simulink subsystem "SurfEngRef"  (R2024b)
settings: Solver=VariableStepAuto  StartTime=0.0  StopTime=10.0  RelTol=1e-3
undefined symbols (not defined in the file): SimIn, SimPar
libraries: simulink x44, ServosLib x5
(part 1 of 2)
settings Model: Creator=drhill  LastModifiedBy=edison
settings SolverCC: AlgebraicLoopSolver=TrustRegion
settings OptimizationCC: ReuseModelBlockBuffer=off
settings DebuggingCC: UnconnectedInputMsg=warning  UnconnectedOutputMsg=warning  UnconnectedLineMsg=warning
settings ModelReferenceCC: EnableRefExpFcnMdlSchedulingChecks=on
settings RTWCC: GPUComputeCapability=3.5  DLArmComputeVersion=19.05

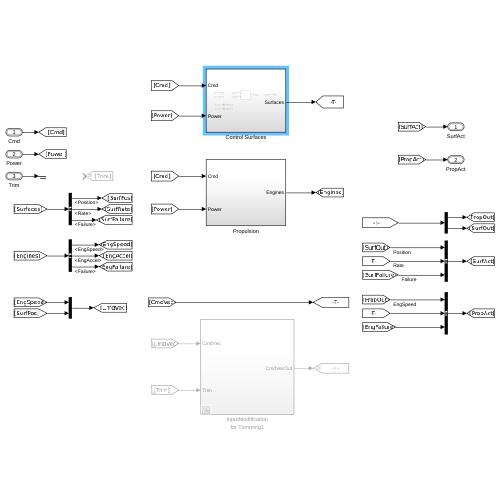
[thumbnail: Simulink's stored preview of the top-level diagram]
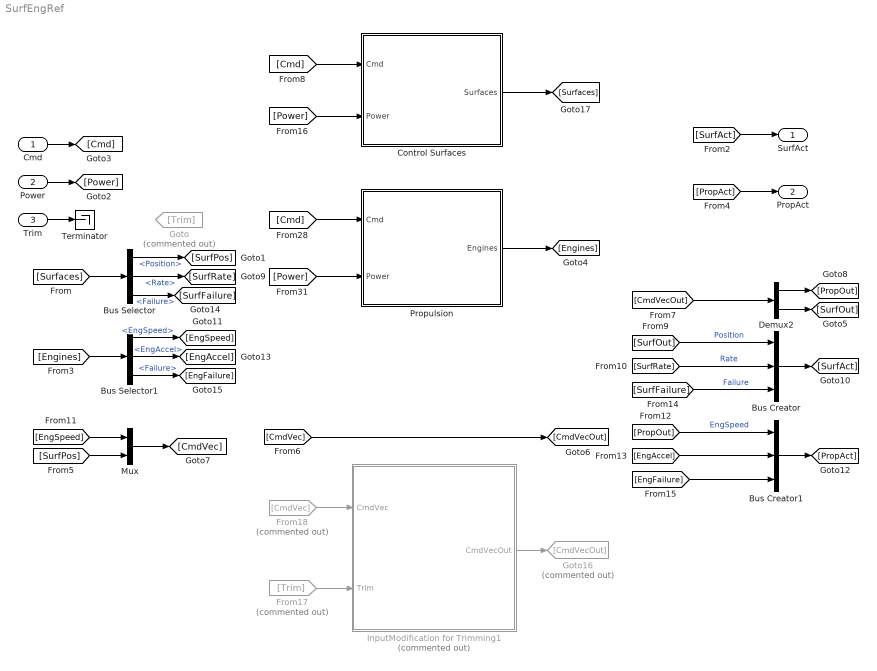
== system SurfEngRef ==
  Cmd : Inport  OutDataTypeStr=Bus: BUS_CMD
  Power : Inport  Port=2  OutDataTypeStr=Bus: BUS_POWER_SYSTEM_OUT
  Trim : Inport  Port=3  OutDataTypeStr=Bus: BUS_TRIM_INPUT
  Bus Creator : BusCreator  Inputs=3  OutDataTypeStr=Bus: BUS_SURF_ACTUATOR
  Bus Creator1 : BusCreator  Inputs=3  OutDataTypeStr=Bus: BUS_PROP_ACTUATOR
  Bus Selector : BusSelector  OutputSignals=Position,Rate,Failure
  Bus Selector1 : BusSelector  OutputSignals=EngSpeed,EngAccel,Failure
  Control Surfaces : Subsystem  VariantControl=GVS_ACT_TYPE_NONE
  Demux2 : Demux  Outputs=[SimIn.numEngines SimIn.numSurfaces]
  From17 : From  Commented=on  GotoTag=Trim
  From18 : From  Commented=on  GotoTag=CmdVec
  Goto : Goto  Commented=on  GotoTag=Trim
  Goto16 : Goto  Commented=on  GotoTag=CmdVecOut
  InputModification for Trimming1 : Subsystem  Commented=on
  Mux : Mux  Inputs=[SimIn.numEngines SimIn.numSurfaces]
  Propulsion : Subsystem  VariantControl=GVS_PROP_TYPE_NONE
  Terminator : Terminator
  SurfAct : Outport  OutDataTypeStr=Bus: BUS_SURF_ACTUATOR
  PropAct : Outport  Port=2  OutDataTypeStr=Bus: BUS_PROP_ACTUATOR
  wires:
  [Cmd] -> Control Surfaces/1(Cmd)
  [Power] -> Control Surfaces/2(Power)
  Control Surfaces/1(Surfaces) -> [Surfaces]
  Trim/1 -> Terminator/1
  Power/1 -> [Power]
  Cmd/1 -> [Cmd]
  [SurfAct] -> SurfAct/1
  [Power] -> Propulsion/2(Power)
  Propulsion/1(Engines) -> [Engines]
  [PropAct] -> PropAct/1
  [Cmd] -> Propulsion/1(Cmd)
  [CmdVec] -> [CmdVecOut]
  Mux/1 -> [CmdVec]
  [CmdVecOut] -> Demux2/1
  Demux2/2 -> [SurfOut]
  Demux2/1 -> [PropOut]
  [Surfaces] -> Bus Selector/1
  Bus Selector/1 -> [SurfPos]  "<Position>"
  [SurfPos] -> Mux/2
  [SurfOut] -> Bus Creator/1  "Position"
  Bus Selector/2 -> [SurfRate]  "<Rate>"
  [SurfRate] -> Bus Creator/2  "Rate"
  Bus Creator/1 -> [SurfAct]
  [Engines] -> Bus Selector1/1
  Bus Selector1/1 -> [EngSpeed]  "<EngSpeed>"
  [EngSpeed] -> Mux/1
  [PropOut] -> Bus Creator1/1  "EngSpeed"
  Bus Creator1/1 -> [PropAct]
  Bus Selector1/2 -> [EngAccel]  "<EngAccel>"
  [EngAccel] -> Bus Creator1/2
  Bus Selector/3 -> [SurfFailure]  "<Failure>"
  [SurfFailure] -> Bus Creator/3  "Failure"
  Bus Selector1/3 -> [EngFailure]  "<Failure>"
  [EngFailure] -> Bus Creator1/3
  InputModification for Trimming1/1(CmdVecOut) -> Goto16/1
  From18/1 -> InputModification for Trimming1/1(CmdVec)
  From17/1 -> InputModification for Trimming1/2(Trim)

== system SurfEngRef/Control Surfaces ==
  Cmd : Inport
  Power : Inport  Port=2
  Bus Selector : BusSelector  OutputSignals=CtrlSurfaceCmd
  Bus Selector1 : BusSelector  OutputSignals=CtrlSurfacePwr
  Control Surface Dynamics : Subsystem  Variant=on
  Surfaces : Outport  VectorParamsAs1DForOutWhenUnconnected=off
  wires:
  [Cmd] -> Bus Selector/1
  Bus Selector/1 -> [SurfCmd]  "<CtrlSurfaceCmd>"
  Bus Selector1/1 -> [SurfPwr]  "<CtrlSurfacePwr>"
  [Power] -> Bus Selector1/1
  [SurfPwr] -> Control Surface Dynamics/2(SurfPwr)
  Control Surface Dynamics/1(SurfAct) -> [SurfAct]
  [SurfCmd] -> Control Surface Dynamics/1(SurfCmd)
  Power/1 -> [Power]
  [SurfAct] -> Surfaces/1
  Cmd/1 -> [Cmd]

== system SurfEngRef/InputModification for Trimming1 ==
  CmdVec : Inport
  Trim : Inport  Port=2  OutDataTypeStr=Bus: BUS_TRIM_INPUT
  Constant : Constant  Value=SimIn.Switches.TrimModeOn
  "Invalid, Error Out" : Subsystem  TreatAsAtomicUnit=on
  Merge : Merge  Inputs=3  InitialOutput=zeros(SimIn.numEngines+SimIn.numSurfaces,1)
  SimMode:PassThrough : Subsystem  TreatAsAtomicUnit=on
  Switch Case : SwitchCase  CaseConditions={0,1}
  TrimMode: DriveFromTopLevel : Subsystem  TreatAsAtomicUnit=on
  CmdVecOut : Outport  VectorParamsAs1DForOutWhenUnconnected=off
  wires:
  [Trim] -> TrimMode: DriveFromTopLevel/1(TrimBias)
  [CmdVec] -> SimMode:PassThrough/1(Cmd)
  Trim/1 -> [Trim]
  CmdVec/1 -> [CmdVec]
  Switch Case/1 -> SimMode:PassThrough/Action
  Switch Case/2 -> TrimMode: DriveFromTopLevel/Action
  SimMode:PassThrough/1(Out) -> Merge/1
  TrimMode: DriveFromTopLevel/1(Out) -> Merge/2
  Merge/1 -> CmdVecOut/1
  Constant/1 -> Switch Case/1
  Switch Case/3 -> "Invalid, Error Out"/Action
  "Invalid, Error Out"/1(Out) -> Merge/3

== system SurfEngRef/Propulsion ==
  Cmd : Inport  OutDataTypeStr=Bus: BUS_CMD
  Power : Inport  Port=2
  Bus Selector : BusSelector  OutputSignals=EngineCmd
  Bus Selector1 : BusSelector  OutputSignals=EnginePwr
  Propulsion Dynamics : Subsystem  Variant=on
  Engines : Outport  OutDataTypeStr=Bus: BUS_PROP_ACTUATOR  VectorParamsAs1DForOutWhenUnconnected=off
  wires:
  Bus Selector1/1 -> [EngPwr]  "<EnginePwr>"
  [Power] -> Bus Selector1/1
  Bus Selector/1 -> [EngCmd]  "<EngineCmd>"
  [Cmd] -> Bus Selector/1
  [EngPwr] -> Propulsion Dynamics/2(EngPwr)
  [EngCmd] -> Propulsion Dynamics/1(EngCmd)
  Propulsion Dynamics/1(PropAct) -> [PropAct]
  [PropAct] -> Engines/1
  Power/1 -> [Power]
  Cmd/1 -> [Cmd]

== system SurfEngRef/Control Surfaces/Control Surface Dynamics ==
  SurfCmd : Inport
  SurfPwr : Inport  Port=2
  FirstOrder : Subsystem  VariantControl=GVS_ACT_TYPE_FIRSTORDER
  FirstOrderFailSurf : Subsystem  VariantControl=GVS_ACT_TYPE_FIRSTORDERFAILSURF
  None : Subsystem  VariantControl=GVS_ACT_TYPE_NONE
  SecondOrder : Subsystem  VariantControl=GVS_ACT_TYPE_SECONDORDER
  SurfAct : Outport

== system SurfEngRef/InputModification for Trimming1/Invalid, Error Out ==
  Action Port : ActionPort
  Constant1 : Constant  Value=zeros(SimIn.numEngines+SimIn.numSurfaces,1)
  Constant2 : Constant  Value=0
  InvalidMode : Assertion  AssertionFailFcn="warndlg('Invalid settings for TrimMode and LinearizeMode.  Run setup.m to reset.','Warning!')"
  Out : Outport  InitialOutput=zeros(SimIn.numEngines+SimIn.numSurfaces,1)  VectorParamsAs1DForOutWhenUnconnected=off
  wires:
  Constant2/1 -> InvalidMode/1
  Constant1/1 -> Out/1

== system SurfEngRef/InputModification for Trimming1/SimMode:PassThrough ==
  Cmd : Inport
  Action Port : ActionPort
  Gain1 : Gain
  Out : Outport  InitialOutput=zeros(SimIn.numEngines+SimIn.numSurfaces,1)  VectorParamsAs1DForOutWhenUnconnected=off
  wires:
  Cmd/1 -> Gain1/1  "LiftEngines(8),TailEngine,Aileron,Flaps,Elevator,Rudder"
  Gain1/1 -> Out/1

== system SurfEngRef/InputModification for Trimming1/TrimMode: DriveFromTopLevel ==
  TrimBias : Inport  OutDataTypeStr=Bus: BUS_TRIM_INPUT
  Action Port : ActionPort
  Bus Selector : BusSelector  OutputSignals=Engines,Surfaces
  Force Consistent Sample Time on Bus : Subsystem  Commented=on
  Multiply : Gain  Gain=SimIn.Trim.surfaceAlloc  Multiplication=Matrix(K*u)
  Mux : Mux  Inputs=2
  Out : Outport  InitialOutput=zeros(SimIn.numEngines+SimIn.numSurfaces,1)  VectorParamsAs1DForOutWhenUnconnected=off
  wires:
  Mux/1 -> Out/1
  Multiply/1 -> Mux/2
  Bus Selector/1 -> Mux/1  "<Engines>"
  TrimBias/1 -> Bus Selector/1
  Bus Selector/2 -> Multiply/1  "<Surfaces>"

== system SurfEngRef/Propulsion/Propulsion Dynamics ==
  EngCmd : Inport
  EngPwr : Inport  Port=2
  FirstOrder : Subsystem  VariantControl=GVS_PROP_TYPE_FIRSTORDER
  FirstOrderFailProp : Subsystem  VariantControl=GVS_PROP_TYPE_FIRSTORDERFAILPROP
  None : Subsystem  VariantControl=GVS_PROP_TYPE_NONE
  SecondOrder : Subsystem  VariantControl=GVS_PROP_TYPE_SECONDORDER
  PropAct : Outport

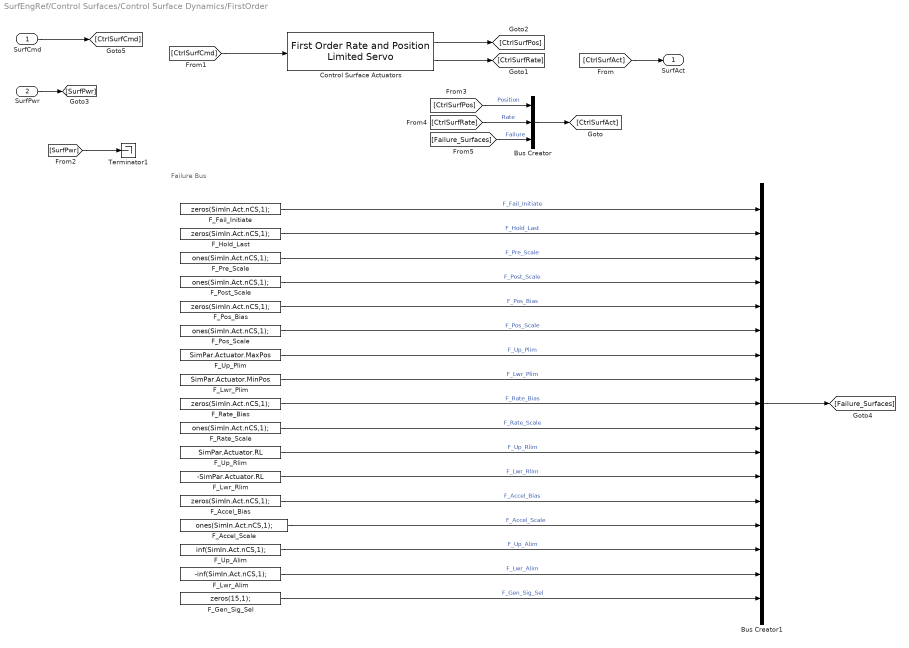
== system SurfEngRef/Control Surfaces/Control Surface Dynamics/FirstOrder ==
  note: Failure Bus
  SurfCmd : Inport
  SurfPwr : Inport  Port=2
  Bus Creator : BusCreator  Inputs=3  OutDataTypeStr=Bus: BUS_SURF_ACTUATOR
  Bus Creator1 : BusCreator  Inputs=17  OutDataTypeStr=Bus: BUS_FAILURE_SURF
  Control Surface Actuators : ServosLib/First Order  Rate and Position Limited  Servo  freq=SimPar.Actuator.BW  RL=SimPar.Actuator.RL  POS_hi=SimPar.Actuator.MaxPos  POS_lo=SimPar.Actuator.MinPos  Bias=SimPar.Actuator.Bias  StateName=Actuators
  F_Accel_Bias : Constant  Value=zeros(SimIn.Act.nCS,1);
  F_Accel_Scale : Constant  Value=ones(SimIn.Act.nCS,1);
  F_Fail_Initiate : Constant  Value=zeros(SimIn.Act.nCS,1);
  F_Gen_Sig_Sel : Constant  Value=zeros(15,1);
  F_Hold_Last : Constant  Value=zeros(SimIn.Act.nCS,1);
  F_Lwr_Alim : Constant  Value=-inf(SimIn.Act.nCS,1);
  F_Lwr_Plim : Constant  Value=SimPar.Actuator.MinPos
  F_Lwr_Rlim : Constant  Value=-SimPar.Actuator.RL
  F_Pos_Bias : Constant  Value=zeros(SimIn.Act.nCS,1);
  F_Pos_Scale : Constant  Value=ones(SimIn.Act.nCS,1);
  F_Post_Scale : Constant  Value=ones(SimIn.Act.nCS,1);
  F_Pre_Scale : Constant  Value=ones(SimIn.Act.nCS,1);
  F_Rate_Bias : Constant  Value=zeros(SimIn.Act.nCS,1);
  F_Rate_Scale : Constant  Value=ones(SimIn.Act.nCS,1);
  F_Up_Alim : Constant  Value=inf(SimIn.Act.nCS,1);
  F_Up_Plim : Constant  Value=SimPar.Actuator.MaxPos
  F_Up_Rlim : Constant  Value=SimPar.Actuator.RL
  Terminator1 : Terminator
  SurfAct : Outport
  wires:
  F_Gen_Sig_Sel/1 -> Bus Creator1/17  "F_Gen_Sig_Sel"
  F_Lwr_Alim/1 -> Bus Creator1/16  "F_Lwr_Alim"
  F_Up_Alim/1 -> Bus Creator1/15  "F_Up_Alim"
  F_Accel_Scale/1 -> Bus Creator1/14  "F_Accel_Scale"
  F_Accel_Bias/1 -> Bus Creator1/13  "F_Accel_Bias"
  F_Lwr_Rlim/1 -> Bus Creator1/12  "F_Lwr_Rlim"
  F_Up_Rlim/1 -> Bus Creator1/11  "F_Up_Rlim"
  F_Rate_Scale/1 -> Bus Creator1/10  "F_Rate_Scale"
  F_Rate_Bias/1 -> Bus Creator1/9  "F_Rate_Bias"
  F_Lwr_Plim/1 -> Bus Creator1/8  "F_Lwr_Plim"
  F_Up_Plim/1 -> Bus Creator1/7  "F_Up_Plim"
  F_Pos_Scale/1 -> Bus Creator1/6  "F_Pos_Scale"
  F_Pos_Bias/1 -> Bus Creator1/5  "F_Pos_Bias"
  F_Post_Scale/1 -> Bus Creator1/4  "F_Post_Scale"
  [Failure_Surfaces] -> Bus Creator/3  "Failure"
  F_Pre_Scale/1 -> Bus Creator1/3  "F_Pre_Scale"
  F_Hold_Last/1 -> Bus Creator1/2  "F_Hold_Last"
  Bus Creator1/1 -> [Failure_Surfaces]
  F_Fail_Initiate/1 -> Bus Creator1/1  "F_Fail_Initiate"
  [SurfPwr] -> Terminator1/1
  SurfPwr/1 -> [SurfPwr]
  SurfCmd/1 -> [CtrlSurfCmd]
  [CtrlSurfCmd] -> Control Surface Actuators/1
  Control Surface Actuators/1 -> [CtrlSurfPos]
  Control Surface Actuators/2 -> [CtrlSurfRate]
  [CtrlSurfAct] -> SurfAct/1
  [CtrlSurfPos] -> Bus Creator/1  "Position"
  [CtrlSurfRate] -> Bus Creator/2  "Rate"
  Bus Creator/1 -> [CtrlSurfAct]

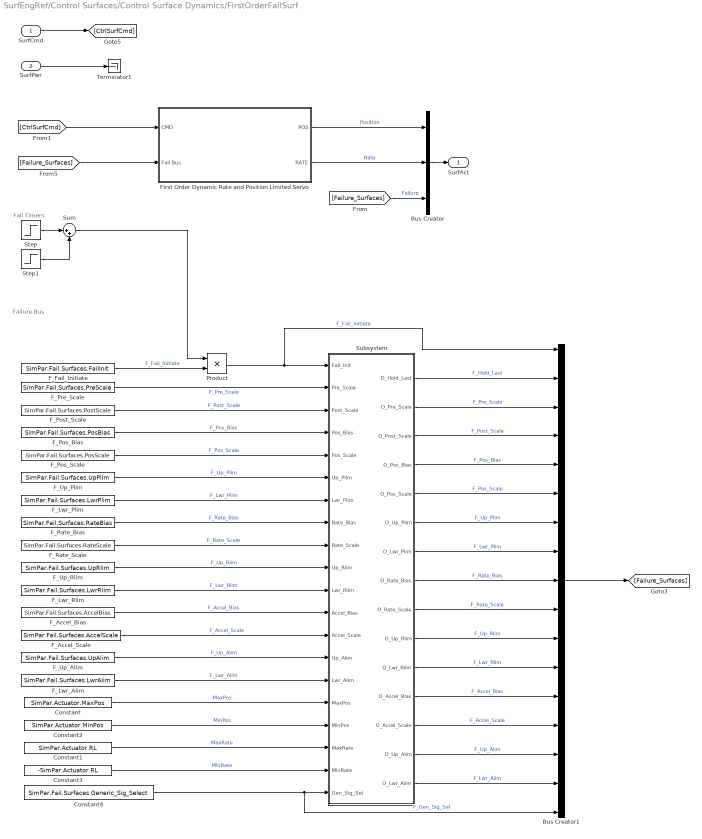
== system SurfEngRef/Control Surfaces/Control Surface Dynamics/FirstOrderFailSurf ==
  note: Failure Bus
  note: Fail Timers
  SurfCmd : Inport
  SurfPwr : Inport  Port=2
  Bus Creator : BusCreator  Inputs=3  OutDataTypeStr=Bus: BUS_SURF_ACTUATOR
  Bus Creator1 : BusCreator  Inputs=17  OutDataTypeStr=Bus: BUS_FAILURE_SURF
  Constant : Constant  Value=SimPar.Actuator.MaxPos
  Constant1 : Constant  Value=SimPar.Actuator.RL
  Constant2 : Constant  Value=SimPar.Actuator.MinPos
  Constant3 : Constant  Value=-SimPar.Actuator.RL
  Constant4 : Constant  Value=SimPar.Fail.Surfaces.Generic_Sig_Select
  F_Accel_Bias : Constant  Value=SimPar.Fail.Surfaces.AccelBias
  F_Accel_Scale : Constant  Value=SimPar.Fail.Surfaces.AccelScale
  F_Fail_Initiate : Constant  Value=SimPar.Fail.Surfaces.FailInit
  F_Lwr_Alim : Constant  Value=SimPar.Fail.Surfaces.LwrAlim
  F_Lwr_Plim : Constant  Value=SimPar.Fail.Surfaces.LwrPlim
  F_Lwr_Rlim : Constant  Value=SimPar.Fail.Surfaces.LwrRlim
  F_Pos_Bias : Constant  Value=SimPar.Fail.Surfaces.PosBias
  F_Pos_Scale : Constant  Value=SimPar.Fail.Surfaces.PosScale
  F_Post_Scale : Constant  Value=SimPar.Fail.Surfaces.PostScale
  F_Pre_Scale : Constant  Value=SimPar.Fail.Surfaces.PreScale
  F_Rate_Bias : Constant  Value=SimPar.Fail.Surfaces.RateBias
  F_Rate_Scale : Constant  Value=SimPar.Fail.Surfaces.RateScale
  F_Up_Alim : Constant  Value=SimPar.Fail.Surfaces.UpAlim
  F_Up_Plim : Constant  Value=SimPar.Fail.Surfaces.UpPlim
  F_Up_Rlim : Constant  Value=SimPar.Fail.Surfaces.UpRlim
  First Order Dynamic Rate and Position Limited Servo : Subsystem  AncestorBlock=ServosLib/First Order Dynamic Rate and Position Limited Servo  mask(Rate and Position Limited Servo){freq=SimPar.Actuator.BW, Bias=SimPar.Actuator.Bias, StateName='Actuators'}
      mask prompts: freq "Bandwidth, Hz:"; Bias "Bias Value, rad:"; StateName "State Name:"
      mask help: First order transfer function: w/(s+w), with rate and position limits and output bias level.
      mask init:
      | %omega=2*pi*freq;
      mask Display:
      | text(.48,.70,'1st Order','horizontalAlignment','center');
      | text(.48,.50,'Rate and Position Limited','horizontalAlignment','center');
      | text(.48,.30,'Filter','horizontalAlignment','center');
  Product : Product
  Step : Step  Time=SimPar.Fail.Surfaces.InitTime  SampleTime=0
  Step1 : Step  Time=SimPar.Fail.Surfaces.StopTime  After=-1  SampleTime=0
  Subsystem : Subsystem
  Sum : Sum  Inputs=|++
  Terminator1 : Terminator
  SurfAct : Outport
  wires:
  [Failure_Surfaces] -> Bus Creator/3  "Failure"
  Constant4/1 -> Bus Creator1/17, Subsystem/20(Gen_Sig_Sel)  "F_Gen_Sig_Sel"
  Sum/1 -> Product/1
  Product/1 -> Subsystem/1(Fail_Init), Bus Creator1/1  "F_Fail_Initiate"
  Step1/1 -> Sum/2
  Step/1 -> Sum/1
  Subsystem/13(O_Accel_Scale) -> Bus Creator1/14  "F_Accel_Scale"
  Subsystem/12(O_Accel_Bias) -> Bus Creator1/13  "F_Accel_Bias"
  Subsystem/15(O_Lwr_Alim) -> Bus Creator1/16  "F_Lwr_Alim"
  Subsystem/14(O_Up_Alim) -> Bus Creator1/15  "F_Up_Alim"
  Subsystem/11(O_Lwr_Rlim) -> Bus Creator1/12  "F_Lwr_Rlim"
  Subsystem/10(O_Up_Rlim) -> Bus Creator1/11  "F_Up_Rlim"
  Subsystem/9(O_Rate_Scale) -> Bus Creator1/10  "F_Rate_Scale"
  Subsystem/8(O_Rate_Bias) -> Bus Creator1/9  "F_Rate_Bias"
  Subsystem/7(O_Lwr_Plim) -> Bus Creator1/8  "F_Lwr_Plim"
  Subsystem/6(O_Up_Plim) -> Bus Creator1/7  "F_Up_Plim"
  Subsystem/5(O_Pos_Scale) -> Bus Creator1/6  "F_Pos_Scale"
  Subsystem/4(O_Pos_Bias) -> Bus Creator1/5  "F_Pos_Bias"
  Subsystem/3(O_Post_Scale) -> Bus Creator1/4  "F_Post_Scale"
  Subsystem/2(O_Pre_Scale) -> Bus Creator1/3  "F_Pre_Scale"
  Subsystem/1(O_Hold_Last) -> Bus Creator1/2  "F_Hold_Last"
  Bus Creator1/1 -> [Failure_Surfaces]
  F_Post_Scale/1 -> Subsystem/3(Post_Scale)  "F_Post_Scale"
  F_Accel_Scale/1 -> Subsystem/13(Accel_Scale)  "F_Accel_Scale"
  F_Lwr_Alim/1 -> Subsystem/15(Lwr_Alim)  "F_Lwr_Alim"
  [Failure_Surfaces] -> First Order Dynamic Rate and Position Limited Servo/2(Fail Bus)
  [CtrlSurfCmd] -> First Order Dynamic Rate and Position Limited Servo/1(CMD)
  First Order Dynamic Rate and Position Limited Servo/2(RATE) -> Bus Creator/2  "Rate"
  F_Lwr_Plim/1 -> Subsystem/7(Lwr_Plim)  "F_Lwr_Plim"
  F_Up_Plim/1 -> Subsystem/6(Up_Plim)  "F_Up_Plim"
  F_Pos_Bias/1 -> Subsystem/4(Pos_Bias)  "F_Pos_Bias"
  F_Rate_Bias/1 -> Subsystem/8(Rate_Bias)  "F_Rate_Bias"
  F_Lwr_Rlim/1 -> Subsystem/11(Lwr_Rlim)  "F_Lwr_Rlim"
  F_Fail_Initiate/1 -> Product/2  "F_Fail_Initiate"
  SurfPwr/1 -> Terminator1/1
  Constant1/1 -> Subsystem/18(MaxRate)  "MaxRate"
  Constant3/1 -> Subsystem/19(MinRate)  "MinRate"
  F_Pos_Scale/1 -> Subsystem/5(Pos_Scale)  "F_Pos_Scale"
  Bus Creator/1 -> SurfAct/1
  Constant2/1 -> Subsystem/17(MinPos)  "MinPos"
  Constant/1 -> Subsystem/16(MaxPos)  "MaxPos"
  F_Pre_Scale/1 -> Subsystem/2(Pre_Scale)  "F_Pre_Scale"
  F_Up_Alim/1 -> Subsystem/14(Up_Alim)  "F_Up_Alim"
  F_Rate_Scale/1 -> Subsystem/9(Rate_Scale)  "F_Rate_Scale"
  F_Accel_Bias/1 -> Subsystem/12(Accel_Bias)  "F_Accel_Bias"
  SurfCmd/1 -> [CtrlSurfCmd]
  F_Up_Rlim/1 -> Subsystem/10(Up_Rlim)  "F_Up_Rlim"
  First Order Dynamic Rate and Position Limited Servo/1(POS) -> Bus Creator/1  "Position"

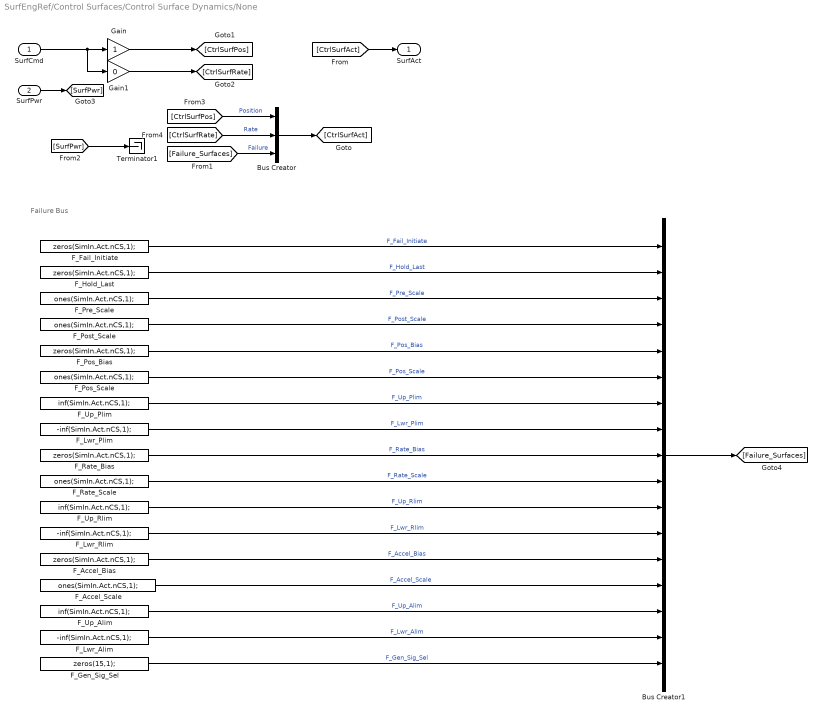
== system SurfEngRef/Control Surfaces/Control Surface Dynamics/None ==
  note: Failure Bus
  SurfCmd : Inport
  SurfPwr : Inport  Port=2
  Bus Creator : BusCreator  Inputs=3  OutDataTypeStr=Bus: BUS_SURF_ACTUATOR
  Bus Creator1 : BusCreator  Inputs=17  OutDataTypeStr=Bus: BUS_FAILURE_SURF
  F_Accel_Bias : Constant  Value=zeros(SimIn.Act.nCS,1);
  F_Accel_Scale : Constant  Value=ones(SimIn.Act.nCS,1);
  F_Fail_Initiate : Constant  Value=zeros(SimIn.Act.nCS,1);
  F_Gen_Sig_Sel : Constant  Value=zeros(15,1);
  F_Hold_Last : Constant  Value=zeros(SimIn.Act.nCS,1);
  F_Lwr_Alim : Constant  Value=-inf(SimIn.Act.nCS,1);
  F_Lwr_Plim : Constant  Value=-inf(SimIn.Act.nCS,1);
  F_Lwr_Rlim : Constant  Value=-inf(SimIn.Act.nCS,1);
  F_Pos_Bias : Constant  Value=zeros(SimIn.Act.nCS,1);
  F_Pos_Scale : Constant  Value=ones(SimIn.Act.nCS,1);
  F_Post_Scale : Constant  Value=ones(SimIn.Act.nCS,1);
  F_Pre_Scale : Constant  Value=ones(SimIn.Act.nCS,1);
  F_Rate_Bias : Constant  Value=zeros(SimIn.Act.nCS,1);
  F_Rate_Scale : Constant  Value=ones(SimIn.Act.nCS,1);
  F_Up_Alim : Constant  Value=inf(SimIn.Act.nCS,1);
  F_Up_Plim : Constant  Value=inf(SimIn.Act.nCS,1);
  F_Up_Rlim : Constant  Value=inf(SimIn.Act.nCS,1);
  Gain : Gain
  Gain1 : Gain  Gain=0
  Terminator1 : Terminator
  SurfAct : Outport
  wires:
  F_Gen_Sig_Sel/1 -> Bus Creator1/17  "F_Gen_Sig_Sel"
  F_Lwr_Alim/1 -> Bus Creator1/16  "F_Lwr_Alim"
  F_Up_Alim/1 -> Bus Creator1/15  "F_Up_Alim"
  F_Accel_Scale/1 -> Bus Creator1/14  "F_Accel_Scale"
  F_Accel_Bias/1 -> Bus Creator1/13  "F_Accel_Bias"
  F_Lwr_Rlim/1 -> Bus Creator1/12  "F_Lwr_Rlim"
  F_Up_Rlim/1 -> Bus Creator1/11  "F_Up_Rlim"
  F_Rate_Scale/1 -> Bus Creator1/10  "F_Rate_Scale"
  F_Rate_Bias/1 -> Bus Creator1/9  "F_Rate_Bias"
  F_Lwr_Plim/1 -> Bus Creator1/8  "F_Lwr_Plim"
  F_Up_Plim/1 -> Bus Creator1/7  "F_Up_Plim"
  F_Pos_Scale/1 -> Bus Creator1/6  "F_Pos_Scale"
  F_Pos_Bias/1 -> Bus Creator1/5  "F_Pos_Bias"
  F_Post_Scale/1 -> Bus Creator1/4  "F_Post_Scale"
  F_Pre_Scale/1 -> Bus Creator1/3  "F_Pre_Scale"
  [Failure_Surfaces] -> Bus Creator/3  "Failure"
  F_Fail_Initiate/1 -> Bus Creator1/1  "F_Fail_Initiate"
  Bus Creator1/1 -> [Failure_Surfaces]
  F_Hold_Last/1 -> Bus Creator1/2  "F_Hold_Last"
  Gain1/1 -> [CtrlSurfRate]
  Gain/1 -> [CtrlSurfPos]
  [CtrlSurfAct] -> SurfAct/1
  [CtrlSurfRate] -> Bus Creator/2  "Rate"
  [CtrlSurfPos] -> Bus Creator/1  "Position"
  Bus Creator/1 -> [CtrlSurfAct]
  [SurfPwr] -> Terminator1/1
  SurfPwr/1 -> [SurfPwr]
  SurfCmd/1 -> Gain1/1, Gain/1

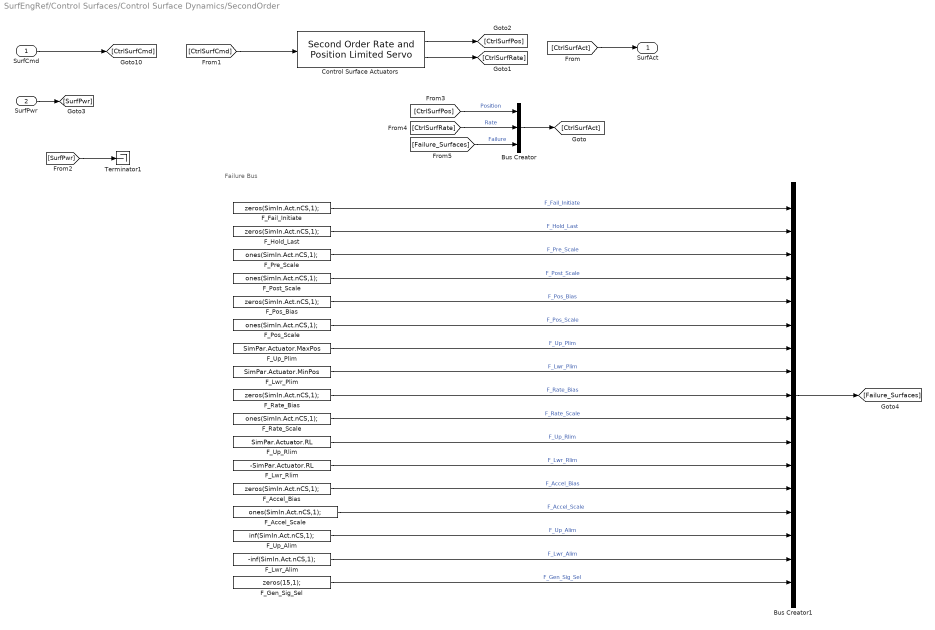
== system SurfEngRef/Control Surfaces/Control Surface Dynamics/SecondOrder ==
  note: Failure Bus
  SurfCmd : Inport
  SurfPwr : Inport  Port=2
  Bus Creator : BusCreator  Inputs=3  OutDataTypeStr=Bus: BUS_SURF_ACTUATOR
  Bus Creator1 : BusCreator  Inputs=17  OutDataTypeStr=Bus: BUS_FAILURE_SURF
  Control Surface Actuators : ServosLib/Second Order Rate and Position Limited Servo  freq=SimPar.Actuator.BW  zeta=SimPar.Actuator.Zeta  RL=SimPar.Actuator.RL  POS_hi=SimPar.Actuator.MaxPos  POS_lo=SimPar.Actuator.MinPos  Bias=SimPar.Actuator.Bias  PosStateName=ActuatorPosition  RateStateName=ActuatorRate
  F_Accel_Bias : Constant  Value=zeros(SimIn.Act.nCS,1);
  F_Accel_Scale : Constant  Value=ones(SimIn.Act.nCS,1);
  F_Fail_Initiate : Constant  Value=zeros(SimIn.Act.nCS,1);
  F_Gen_Sig_Sel : Constant  Value=zeros(15,1);
  F_Hold_Last : Constant  Value=zeros(SimIn.Act.nCS,1);
  F_Lwr_Alim : Constant  Value=-inf(SimIn.Act.nCS,1);
  F_Lwr_Plim : Constant  Value=SimPar.Actuator.MinPos
  F_Lwr_Rlim : Constant  Value=-SimPar.Actuator.RL
  F_Pos_Bias : Constant  Value=zeros(SimIn.Act.nCS,1);
  F_Pos_Scale : Constant  Value=ones(SimIn.Act.nCS,1);
  F_Post_Scale : Constant  Value=ones(SimIn.Act.nCS,1);
  F_Pre_Scale : Constant  Value=ones(SimIn.Act.nCS,1);
  F_Rate_Bias : Constant  Value=zeros(SimIn.Act.nCS,1);
  F_Rate_Scale : Constant  Value=ones(SimIn.Act.nCS,1);
  F_Up_Alim : Constant  Value=inf(SimIn.Act.nCS,1);
  F_Up_Plim : Constant  Value=SimPar.Actuator.MaxPos
  F_Up_Rlim : Constant  Value=SimPar.Actuator.RL
  Terminator1 : Terminator
  SurfAct : Outport
  wires:
  F_Lwr_Alim/1 -> Bus Creator1/16  "F_Lwr_Alim"
  F_Rate_Scale/1 -> Bus Creator1/10  "F_Rate_Scale"
  F_Rate_Bias/1 -> Bus Creator1/9  "F_Rate_Bias"
  F_Post_Scale/1 -> Bus Creator1/4  "F_Post_Scale"
  F_Up_Rlim/1 -> Bus Creator1/11  "F_Up_Rlim"
  F_Lwr_Rlim/1 -> Bus Creator1/12  "F_Lwr_Rlim"
  F_Hold_Last/1 -> Bus Creator1/2  "F_Hold_Last"
  F_Lwr_Plim/1 -> Bus Creator1/8  "F_Lwr_Plim"
  F_Accel_Bias/1 -> Bus Creator1/13  "F_Accel_Bias"
  F_Gen_Sig_Sel/1 -> Bus Creator1/17  "F_Gen_Sig_Sel"
  F_Accel_Scale/1 -> Bus Creator1/14  "F_Accel_Scale"
  F_Up_Alim/1 -> Bus Creator1/15  "F_Up_Alim"
  F_Pre_Scale/1 -> Bus Creator1/3  "F_Pre_Scale"
  F_Up_Plim/1 -> Bus Creator1/7  "F_Up_Plim"
  F_Pos_Bias/1 -> Bus Creator1/5  "F_Pos_Bias"
  F_Pos_Scale/1 -> Bus Creator1/6  "F_Pos_Scale"
  F_Fail_Initiate/1 -> Bus Creator1/1  "F_Fail_Initiate"
  Bus Creator1/1 -> [Failure_Surfaces]
  [Failure_Surfaces] -> Bus Creator/3  "Failure"
  [CtrlSurfRate] -> Bus Creator/2  "Rate"
  [CtrlSurfPos] -> Bus Creator/1  "Position"
  Bus Creator/1 -> [CtrlSurfAct]
  Control Surface Actuators/2 -> [CtrlSurfRate]
  Control Surface Actuators/1 -> [CtrlSurfPos]
  [SurfPwr] -> Terminator1/1
  SurfCmd/1 -> [CtrlSurfCmd]
  [CtrlSurfCmd] -> Control Surface Actuators/1
  [CtrlSurfAct] -> SurfAct/1
  SurfPwr/1 -> [SurfPwr]

== system SurfEngRef/InputModification for Trimming1/TrimMode: DriveFromTopLevel/Force Consistent Sample Time on Bus ==
  TrimBias : Inport
  Bus to Vector : BusToVector
  Map4 : Gain
  Out1 : Outport  VectorParamsAs1DForOutWhenUnconnected=off
  wires:
  Bus to Vector/1 -> Map4/1
  Map4/1 -> Out1/1
  TrimBias/1 -> Bus to Vector/1

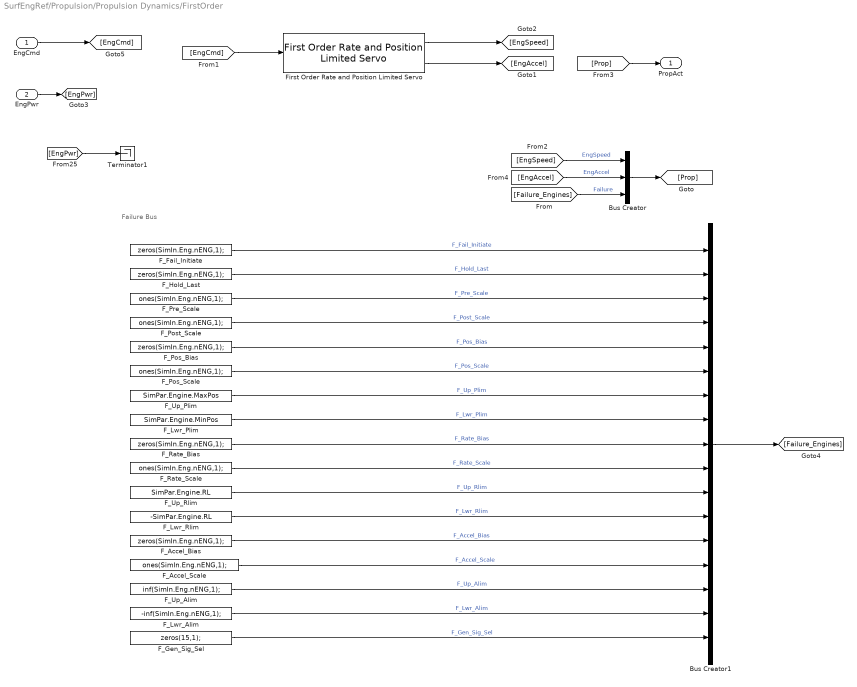
== system SurfEngRef/Propulsion/Propulsion Dynamics/FirstOrder ==
  note: Failure Bus
  EngCmd : Inport
  EngPwr : Inport  Port=2
  Bus Creator : BusCreator  Inputs=3  OutDataTypeStr=Bus: BUS_PROP_ACTUATOR
  Bus Creator1 : BusCreator  Inputs=17  OutDataTypeStr=Bus: BUS_FAILURE_ENG
  F_Accel_Bias : Constant  Value=zeros(SimIn.Eng.nENG,1);
  F_Accel_Scale : Constant  Value=ones(SimIn.Eng.nENG,1);
  F_Fail_Initiate : Constant  Value=zeros(SimIn.Eng.nENG,1);
  F_Gen_Sig_Sel : Constant  Value=zeros(15,1);
  F_Hold_Last : Constant  Value=zeros(SimIn.Eng.nENG,1);
  F_Lwr_Alim : Constant  Value=-inf(SimIn.Eng.nENG,1);
  F_Lwr_Plim : Constant  Value=SimPar.Engine.MinPos
  F_Lwr_Rlim : Constant  Value=-SimPar.Engine.RL
  F_Pos_Bias : Constant  Value=zeros(SimIn.Eng.nENG,1);
  F_Pos_Scale : Constant  Value=ones(SimIn.Eng.nENG,1);
  F_Post_Scale : Constant  Value=ones(SimIn.Eng.nENG,1);
  F_Pre_Scale : Constant  Value=ones(SimIn.Eng.nENG,1);
  F_Rate_Bias : Constant  Value=zeros(SimIn.Eng.nENG,1);
  F_Rate_Scale : Constant  Value=ones(SimIn.Eng.nENG,1);
  F_Up_Alim : Constant  Value=inf(SimIn.Eng.nENG,1);
  F_Up_Plim : Constant  Value=SimPar.Engine.MaxPos
  F_Up_Rlim : Constant  Value=SimPar.Engine.RL
  First Order Rate and Position Limited Servo : ServosLib/First Order  Rate and Position Limited  Servo  freq=SimPar.Engine.BW  RL=SimPar.Engine.RL  POS_hi=SimPar.Engine.MaxPos  POS_lo=SimPar.Engine.MinPos  Bias=SimPar.Engine.Bias  StateName=EngineSpeed
  Terminator1 : Terminator
  PropAct : Outport
  wires:
  [Failure_Engines] -> Bus Creator/3  "Failure"
  F_Lwr_Alim/1 -> Bus Creator1/16  "F_Lwr_Alim"
  F_Rate_Scale/1 -> Bus Creator1/10  "F_Rate_Scale"
  F_Rate_Bias/1 -> Bus Creator1/9  "F_Rate_Bias"
  F_Post_Scale/1 -> Bus Creator1/4  "F_Post_Scale"
  F_Up_Rlim/1 -> Bus Creator1/11  "F_Up_Rlim"
  F_Lwr_Rlim/1 -> Bus Creator1/12  "F_Lwr_Rlim"
  F_Hold_Last/1 -> Bus Creator1/2  "F_Hold_Last"
  F_Lwr_Plim/1 -> Bus Creator1/8  "F_Lwr_Plim"
  F_Accel_Bias/1 -> Bus Creator1/13  "F_Accel_Bias"
  F_Gen_Sig_Sel/1 -> Bus Creator1/17  "F_Gen_Sig_Sel"
  F_Accel_Scale/1 -> Bus Creator1/14  "F_Accel_Scale"
  F_Up_Alim/1 -> Bus Creator1/15  "F_Up_Alim"
  F_Pre_Scale/1 -> Bus Creator1/3  "F_Pre_Scale"
  F_Up_Plim/1 -> Bus Creator1/7  "F_Up_Plim"
  F_Pos_Bias/1 -> Bus Creator1/5  "F_Pos_Bias"
  F_Pos_Scale/1 -> Bus Creator1/6  "F_Pos_Scale"
  F_Fail_Initiate/1 -> Bus Creator1/1  "F_Fail_Initiate"
  Bus Creator1/1 -> [Failure_Engines]
  First Order Rate and Position Limited Servo/2 -> [EngAccel]
  First Order Rate and Position Limited Servo/1 -> [EngSpeed]
  [Prop] -> PropAct/1
  [EngPwr] -> Terminator1/1
  [EngCmd] -> First Order Rate and Position Limited Servo/1
  EngPwr/1 -> [EngPwr]
  EngCmd/1 -> [EngCmd]
  [EngSpeed] -> Bus Creator/1  "EngSpeed"
  Bus Creator/1 -> [Prop]
  [EngAccel] -> Bus Creator/2  "EngAccel"

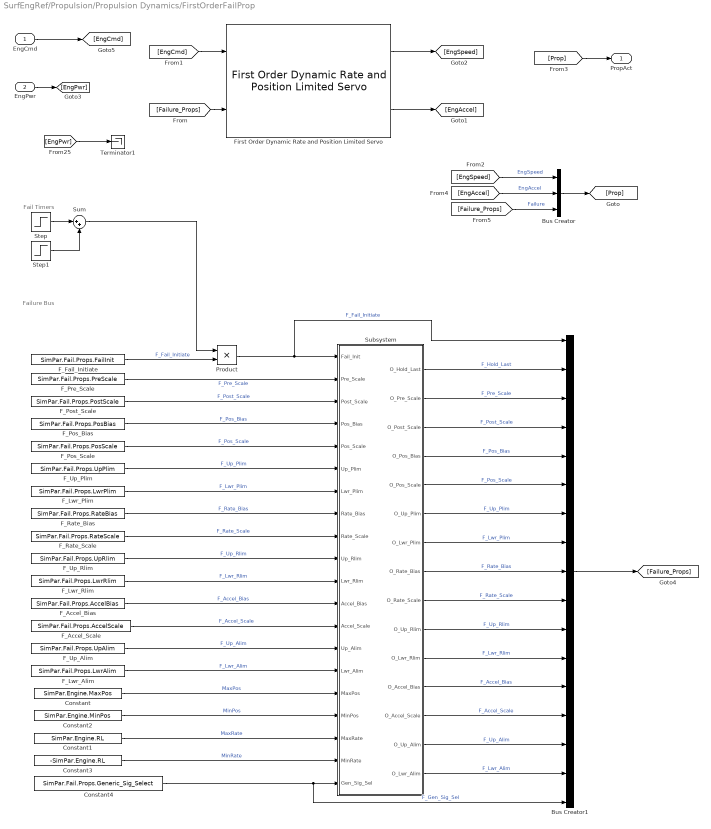
== system SurfEngRef/Propulsion/Propulsion Dynamics/FirstOrderFailProp ==
  note: Failure Bus
  note: Fail Timers
  EngCmd : Inport
  EngPwr : Inport  Port=2
  Bus Creator : BusCreator  Inputs=3  OutDataTypeStr=Bus: BUS_PROP_ACTUATOR
  Bus Creator1 : BusCreator  Inputs=17  OutDataTypeStr=Bus: BUS_FAILURE_ENG
  Constant : Constant  Value=SimPar.Engine.MaxPos
  Constant1 : Constant  Value=SimPar.Engine.RL
  Constant2 : Constant  Value=SimPar.Engine.MinPos
  Constant3 : Constant  Value=-SimPar.Engine.RL
  Constant4 : Constant  Value=SimPar.Fail.Props.Generic_Sig_Select
  F_Accel_Bias : Constant  Value=SimPar.Fail.Props.AccelBias
  F_Accel_Scale : Constant  Value=SimPar.Fail.Props.AccelScale
  F_Fail_Initiate : Constant  Value=SimPar.Fail.Props.FailInit
  F_Lwr_Alim : Constant  Value=SimPar.Fail.Props.LwrAlim
  F_Lwr_Plim : Constant  Value=SimPar.Fail.Props.LwrPlim
  F_Lwr_Rlim : Constant  Value=SimPar.Fail.Props.LwrRlim
  F_Pos_Bias : Constant  Value=SimPar.Fail.Props.PosBias
  F_Pos_Scale : Constant  Value=SimPar.Fail.Props.PosScale
  F_Post_Scale : Constant  Value=SimPar.Fail.Props.PostScale
  F_Pre_Scale : Constant  Value=SimPar.Fail.Props.PreScale
  F_Rate_Bias : Constant  Value=SimPar.Fail.Props.RateBias
  F_Rate_Scale : Constant  Value=SimPar.Fail.Props.RateScale
  F_Up_Alim : Constant  Value=SimPar.Fail.Props.UpAlim
  F_Up_Plim : Constant  Value=SimPar.Fail.Props.UpPlim
  F_Up_Rlim : Constant  Value=SimPar.Fail.Props.UpRlim
  First Order Dynamic Rate and Position Limited Servo : ServosLib/First Order Dynamic Rate and Position Limited Servo  freq=SimPar.Engine.BW  Bias=SimPar.Engine.Bias  StateName='Engines'
  Product : Product
  Step : Step  Time=SimPar.Fail.Props.InitTime  SampleTime=0
  Step1 : Step  Time=SimPar.Fail.Props.StopTime  After=-1  SampleTime=0
  Subsystem : Subsystem
  Sum : Sum  Inputs=|++
  Terminator1 : Terminator
  PropAct : Outport
  wires:
  [EngPwr] -> Terminator1/1
  [EngAccel] -> Bus Creator/2  "EngAccel"
  Bus Creator/1 -> [Prop]
  First Order Dynamic Rate and Position Limited Servo/2 -> [EngAccel]
  [Prop] -> PropAct/1
  [EngSpeed] -> Bus Creator/1  "EngSpeed"
  EngPwr/1 -> [EngPwr]
  EngCmd/1 -> [EngCmd]
  [EngCmd] -> First Order Dynamic Rate and Position Limited Servo/1
  First Order Dynamic Rate and Position Limited Servo/1 -> [EngSpeed]
  F_Up_Rlim/1 -> Subsystem/10(Up_Rlim)  "F_Up_Rlim"
  Subsystem/4(O_Pos_Bias) -> Bus Creator1/5  "F_Pos_Bias"
  F_Accel_Bias/1 -> Subsystem/12(Accel_Bias)  "F_Accel_Bias"
  Subsystem/11(O_Lwr_Rlim) -> Bus Creator1/12  "F_Lwr_Rlim"
  F_Pos_Bias/1 -> Subsystem/4(Pos_Bias)  "F_Pos_Bias"
  F_Rate_Bias/1 -> Subsystem/8(Rate_Bias)  "F_Rate_Bias"
  Constant2/1 -> Subsystem/17(MinPos)  "MinPos"
  F_Up_Alim/1 -> Subsystem/14(Up_Alim)  "F_Up_Alim"
  Product/1 -> Subsystem/1(Fail_Init), Bus Creator1/1  "F_Fail_Initiate"
  F_Pre_Scale/1 -> Subsystem/2(Pre_Scale)  "F_Pre_Scale"
  F_Pos_Scale/1 -> Subsystem/5(Pos_Scale)  "F_Pos_Scale"
  F_Fail_Initiate/1 -> Product/2  "F_Fail_Initiate"
  Subsystem/13(O_Accel_Scale) -> Bus Creator1/14  "F_Accel_Scale"
  F_Rate_Scale/1 -> Subsystem/9(Rate_Scale)  "F_Rate_Scale"
  Constant1/1 -> Subsystem/18(MaxRate)  "MaxRate"
  F_Lwr_Rlim/1 -> Subsystem/11(Lwr_Rlim)  "F_Lwr_Rlim"
  F_Lwr_Plim/1 -> Subsystem/7(Lwr_Plim)  "F_Lwr_Plim"
  Subsystem/12(O_Accel_Bias) -> Bus Creator1/13  "F_Accel_Bias"
  Constant3/1 -> Subsystem/19(MinRate)  "MinRate"
  Subsystem/5(O_Pos_Scale) -> Bus Creator1/6  "F_Pos_Scale"
  Subsystem/2(O_Pre_Scale) -> Bus Creator1/3  "F_Pre_Scale"
  Subsystem/7(O_Lwr_Plim) -> Bus Creator1/8  "F_Lwr_Plim"
  F_Accel_Scale/1 -> Subsystem/13(Accel_Scale)  "F_Accel_Scale"
  F_Post_Scale/1 -> Subsystem/3(Post_Scale)  "F_Post_Scale"
  Subsystem/14(O_Up_Alim) -> Bus Creator1/15  "F_Up_Alim"
  F_Lwr_Alim/1 -> Subsystem/15(Lwr_Alim)  "F_Lwr_Alim"
  Step/1 -> Sum/1
  Subsystem/10(O_Up_Rlim) -> Bus Creator1/11  "F_Up_Rlim"
  Bus Creator1/1 -> [Failure_Props]
  Subsystem/6(O_Up_Plim) -> Bus Creator1/7  "F_Up_Plim"
  Subsystem/8(O_Rate_Bias) -> Bus Creator1/9  "F_Rate_Bias"
  Constant4/1 -> Bus Creator1/17, Subsystem/20(Gen_Sig_Sel)  "F_Gen_Sig_Sel"
  F_Up_Plim/1 -> Subsystem/6(Up_Plim)  "F_Up_Plim"
  Step1/1 -> Sum/2
  Subsystem/15(O_Lwr_Alim) -> Bus Creator1/16  "F_Lwr_Alim"
  Constant/1 -> Subsystem/16(MaxPos)  "MaxPos"
  Subsystem/1(O_Hold_Last) -> Bus Creator1/2  "F_Hold_Last"
  Sum/1 -> Product/1
  Subsystem/3(O_Post_Scale) -> Bus Creator1/4  "F_Post_Scale"
  Subsystem/9(O_Rate_Scale) -> Bus Creator1/10  "F_Rate_Scale"
  [Failure_Props] -> First Order Dynamic Rate and Position Limited Servo/2
  [Failure_Props] -> Bus Creator/3  "Failure"

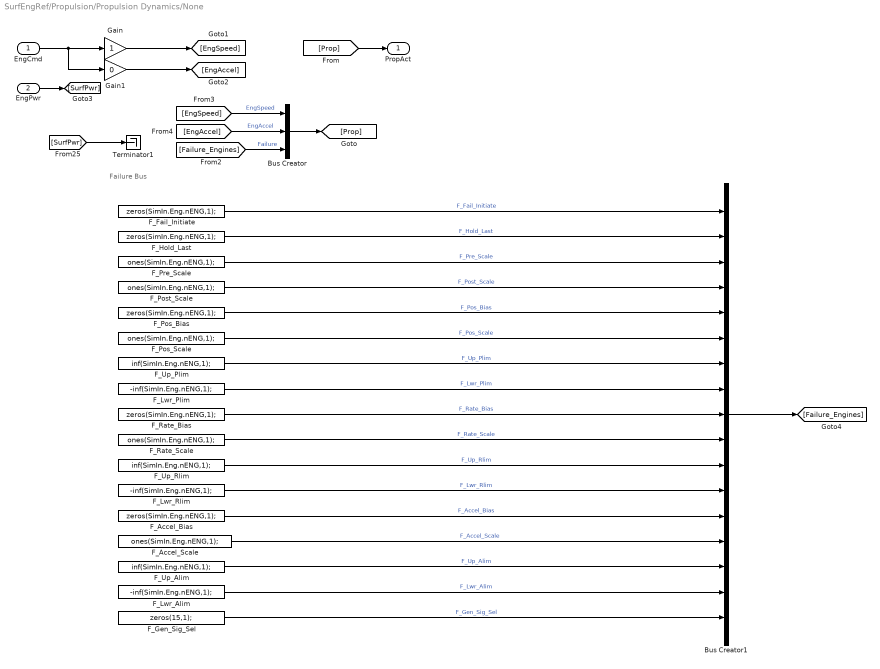
== system SurfEngRef/Propulsion/Propulsion Dynamics/None ==
  note: Failure Bus
  EngCmd : Inport
  EngPwr : Inport  Port=2
  Bus Creator : BusCreator  Inputs=3  OutDataTypeStr=Bus: BUS_PROP_ACTUATOR
  Bus Creator1 : BusCreator  Inputs=17  OutDataTypeStr=Bus: BUS_FAILURE_ENG
  F_Accel_Bias : Constant  Value=zeros(SimIn.Eng.nENG,1);
  F_Accel_Scale : Constant  Value=ones(SimIn.Eng.nENG,1);
  F_Fail_Initiate : Constant  Value=zeros(SimIn.Eng.nENG,1);
  F_Gen_Sig_Sel : Constant  Value=zeros(15,1);
  F_Hold_Last : Constant  Value=zeros(SimIn.Eng.nENG,1);
  F_Lwr_Alim : Constant  Value=-inf(SimIn.Eng.nENG,1);
  F_Lwr_Plim : Constant  Value=-inf(SimIn.Eng.nENG,1);
  F_Lwr_Rlim : Constant  Value=-inf(SimIn.Eng.nENG,1);
  F_Pos_Bias : Constant  Value=zeros(SimIn.Eng.nENG,1);
  F_Pos_Scale : Constant  Value=ones(SimIn.Eng.nENG,1);
  F_Post_Scale : Constant  Value=ones(SimIn.Eng.nENG,1);
  F_Pre_Scale : Constant  Value=ones(SimIn.Eng.nENG,1);
  F_Rate_Bias : Constant  Value=zeros(SimIn.Eng.nENG,1);
  F_Rate_Scale : Constant  Value=ones(SimIn.Eng.nENG,1);
  F_Up_Alim : Constant  Value=inf(SimIn.Eng.nENG,1);
  F_Up_Plim : Constant  Value=inf(SimIn.Eng.nENG,1);
  F_Up_Rlim : Constant  Value=inf(SimIn.Eng.nENG,1);
  Gain : Gain
  Gain1 : Gain  Gain=0
  Terminator1 : Terminator
  PropAct : Outport
  wires:
  [Failure_Engines] -> Bus Creator/3  "Failure"
  F_Fail_Initiate/1 -> Bus Creator1/1  "F_Fail_Initiate"
  Bus Creator1/1 -> [Failure_Engines]
  F_Rate_Scale/1 -> Bus Creator1/10  "F_Rate_Scale"
  F_Up_Rlim/1 -> Bus Creator1/11  "F_Up_Rlim"
  F_Lwr_Plim/1 -> Bus Creator1/8  "F_Lwr_Plim"
  F_Pre_Scale/1 -> Bus Creator1/3  "F_Pre_Scale"
  F_Pos_Scale/1 -> Bus Creator1/6  "F_Pos_Scale"
  F_Rate_Bias/1 -> Bus Creator1/9  "F_Rate_Bias"
  F_Accel_Bias/1 -> Bus Creator1/13  "F_Accel_Bias"
  F_Hold_Last/1 -> Bus Creator1/2  "F_Hold_Last"
  F_Lwr_Rlim/1 -> Bus Creator1/12  "F_Lwr_Rlim"
  F_Lwr_Alim/1 -> Bus Creator1/16  "F_Lwr_Alim"
  F_Post_Scale/1 -> Bus Creator1/4  "F_Post_Scale"
  F_Accel_Scale/1 -> Bus Creator1/14  "F_Accel_Scale"
  F_Pos_Bias/1 -> Bus Creator1/5  "F_Pos_Bias"
  F_Up_Plim/1 -> Bus Creator1/7  "F_Up_Plim"
  F_Up_Alim/1 -> Bus Creator1/15  "F_Up_Alim"
  F_Gen_Sig_Sel/1 -> Bus Creator1/17  "F_Gen_Sig_Sel"
  Gain1/1 -> [EngAccel]
  [Prop] -> PropAct/1
  [EngAccel] -> Bus Creator/2  "EngAccel"
  [EngSpeed] -> Bus Creator/1  "EngSpeed"
  [SurfPwr] -> Terminator1/1
  EngPwr/1 -> [SurfPwr]
  EngCmd/1 -> Gain/1, Gain1/1
  Bus Creator/1 -> [Prop]
  Gain/1 -> [EngSpeed]

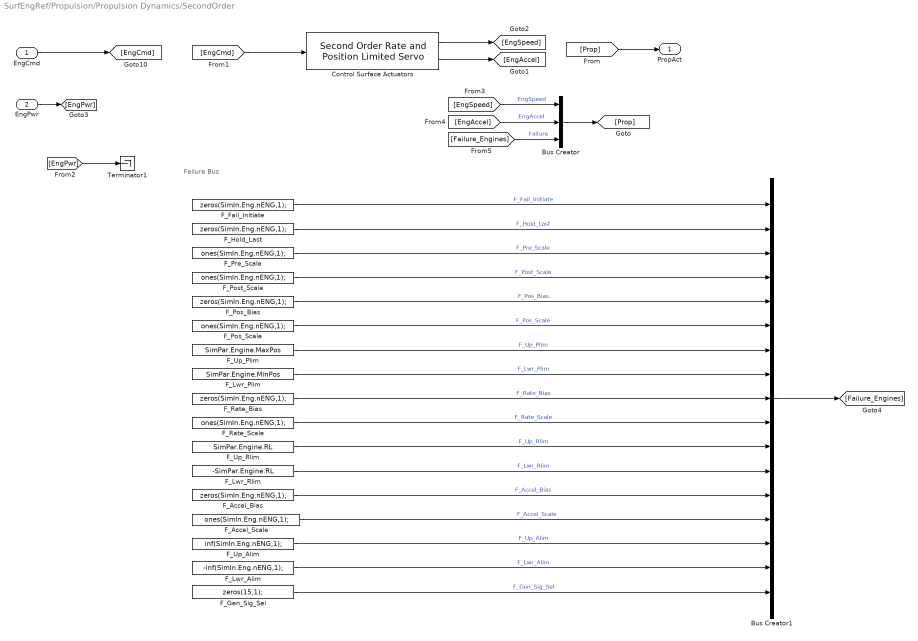
== system SurfEngRef/Propulsion/Propulsion Dynamics/SecondOrder ==
  note: Failure Bus
  EngCmd : Inport
  EngPwr : Inport  Port=2
  Bus Creator : BusCreator  Inputs=3  OutDataTypeStr=Bus: BUS_PROP_ACTUATOR
  Bus Creator1 : BusCreator  Inputs=17  OutDataTypeStr=Bus: BUS_FAILURE_ENG
  Control Surface Actuators : ServosLib/Second Order Rate and Position Limited Servo  freq=SimPar.Engine.BW  zeta=SimPar.Engine.Zeta  RL=SimPar.Engine.RL  POS_hi=SimPar.Engine.MaxPos  POS_lo=SimPar.Engine.MinPos  Bias=SimPar.Engine.Bias  PosStateName=EngineSpeed  RateStateName=EngineAccel
  F_Accel_Bias : Constant  Value=zeros(SimIn.Eng.nENG,1);
  F_Accel_Scale : Constant  Value=ones(SimIn.Eng.nENG,1);
  F_Fail_Initiate : Constant  Value=zeros(SimIn.Eng.nENG,1);
  F_Gen_Sig_Sel : Constant  Value=zeros(15,1);
  F_Hold_Last : Constant  Value=zeros(SimIn.Eng.nENG,1);
  F_Lwr_Alim : Constant  Value=-inf(SimIn.Eng.nENG,1);
  F_Lwr_Plim : Constant  Value=SimPar.Engine.MinPos
  F_Lwr_Rlim : Constant  Value=-SimPar.Engine.RL
  F_Pos_Bias : Constant  Value=zeros(SimIn.Eng.nENG,1);
  F_Pos_Scale : Constant  Value=ones(SimIn.Eng.nENG,1);
  F_Post_Scale : Constant  Value=ones(SimIn.Eng.nENG,1);
  F_Pre_Scale : Constant  Value=ones(SimIn.Eng.nENG,1);
  F_Rate_Bias : Constant  Value=zeros(SimIn.Eng.nENG,1);
  F_Rate_Scale : Constant  Value=ones(SimIn.Eng.nENG,1);
  F_Up_Alim : Constant  Value=inf(SimIn.Eng.nENG,1);
  F_Up_Plim : Constant  Value=SimPar.Engine.MaxPos
  F_Up_Rlim : Constant  Value=SimPar.Engine.RL
  Terminator1 : Terminator
  PropAct : Outport
  wires:
  [Failure_Engines] -> Bus Creator/3  "Failure"
  F_Up_Alim/1 -> Bus Creator1/15  "F_Up_Alim"
  F_Pos_Scale/1 -> Bus Creator1/6  "F_Pos_Scale"
  F_Fail_Initiate/1 -> Bus Creator1/1  "F_Fail_Initiate"
  Bus Creator1/1 -> [Failure_Engines]
  F_Pos_Bias/1 -> Bus Creator1/5  "F_Pos_Bias"
  F_Hold_Last/1 -> Bus Creator1/2  "F_Hold_Last"
  F_Up_Plim/1 -> Bus Creator1/7  "F_Up_Plim"
  F_Pre_Scale/1 -> Bus Creator1/3  "F_Pre_Scale"
  F_Gen_Sig_Sel/1 -> Bus Creator1/17  "F_Gen_Sig_Sel"
  F_Accel_Bias/1 -> Bus Creator1/13  "F_Accel_Bias"
  F_Lwr_Plim/1 -> Bus Creator1/8  "F_Lwr_Plim"
  F_Accel_Scale/1 -> Bus Creator1/14  "F_Accel_Scale"
  F_Up_Rlim/1 -> Bus Creator1/11  "F_Up_Rlim"
  F_Post_Scale/1 -> Bus Creator1/4  "F_Post_Scale"
  F_Rate_Bias/1 -> Bus Creator1/9  "F_Rate_Bias"
  F_Lwr_Rlim/1 -> Bus Creator1/12  "F_Lwr_Rlim"
  F_Rate_Scale/1 -> Bus Creator1/10  "F_Rate_Scale"
  F_Lwr_Alim/1 -> Bus Creator1/16  "F_Lwr_Alim"
  EngPwr/1 -> [EngPwr]
  [Prop] -> PropAct/1
  [EngCmd] -> Control Surface Actuators/1
  EngCmd/1 -> [EngCmd]
  [EngPwr] -> Terminator1/1
  Control Surface Actuators/1 -> [EngSpeed]
  Control Surface Actuators/2 -> [EngAccel]
  Bus Creator/1 -> [Prop]
  [EngSpeed] -> Bus Creator/1  "EngSpeed"
  [EngAccel] -> Bus Creator/2  "EngAccel"

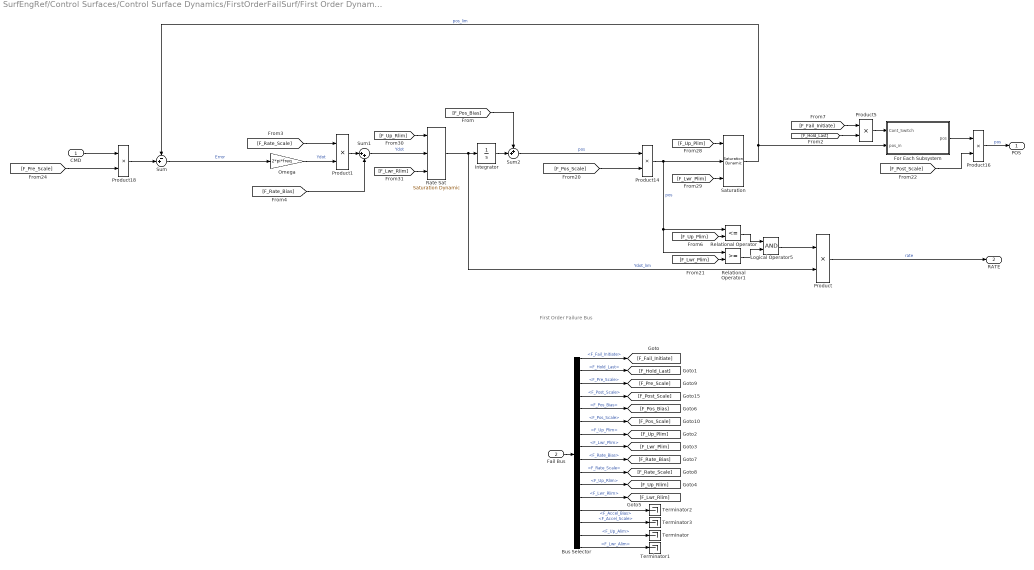
== system SurfEngRef/Control Surfaces/Control Surface Dynamics/FirstOrderFailSurf/First Order Dynamic Rate and Position Limited Servo ==
  note: First Order Failure Bus
  CMD : Inport
  Fail Bus : Inport  Port=2
  Bus Selector : BusSelector  OutputSignals=F_Fail_Initiate,F_Hold_Last,F_Pre_Scale,F_Post_Scale,F_Pos_Bias,F_Pos_Scale,F_Up_Plim,F_Lwr_Plim,F_Rate_Bias,F_Rate_Scale,F_Up_Rlim,F_Lwr_Rlim,F_Accel_Bias,F_Accel_Scale,F_Up_Alim,F_Lwr_Alim
  For Each Subsystem : Subsystem  TreatAsAtomicUnit=on
  Integrator : Integrator  InitialCondition=Bias  LimitOutput=on  UpperSaturationLimit=SimIn.Act.PosLim_hi  LowerSaturationLimit=SimIn.Act.PosLim_lo  IgnoreLimit=on  ContinuousStateAttributes=StateName
  Logical Operator5 : Logic  AllPortsSameDT=off  OutDataTypeStr=boolean
  Omega : Gain  Gain=2*pi*freq  SaturateOnIntegerOverflow=on  OutDataTypeStr=Inherit: Same as input  ParamDataTypeStr=Inherit: Same as input
  Product : Product  RndMeth=Zero
  Product{1,5,14,16,18} (5 alike) : Product
  Rate Sat : simulink/Discontinuities/Saturation Dynamic  OutMin=[]  OutMax=[]  OutDataTypeStr=Inherit: Same as second input  OutDataType=fixdt(1, 16)  OutScaling=2^-10  DoSatur=off
  Relational Operator : RelationalOperator  Operator=<=  OutDataTypeStr=boolean  RndMeth=Simplest  InputSameDT=off
  Relational Operator1 : RelationalOperator  OutDataTypeStr=boolean  RndMeth=Simplest  InputSameDT=off
  Saturation : simulink/Discontinuities/Saturation Dynamic  OutMin=[]  OutMax=[]  OutDataTypeStr=Inherit: Same as second input  OutDataType=fixdt(1, 16)  OutScaling=2^-10  DoSatur=off
  Sum : Sum  Inputs=-+|  InputSameDT=on  SaturateOnIntegerOverflow=on  OutDataTypeStr=Inherit: Same as first input
  Sum1 : Sum  Inputs=|++  InputSameDT=on  SaturateOnIntegerOverflow=on  OutDataTypeStr=Inherit: Same as first input
  Sum2 : Sum  Inputs=++|
  Terminator{,1..3} (4 alike) : Terminator
  POS : Outport  VectorParamsAs1DForOutWhenUnconnected=off
  RATE : Outport  Port=2
  wires:
  CMD/1 -> Product18/1
  Rate Sat/1 -> Product/2, Integrator/1  "Ydot_lim"
  Sum/1 -> Omega/1  "Error"
  Omega/1 -> Product1/2  "Ydot"
  Product/1 -> RATE/1  "rate"
  Fail Bus/1 -> Bus Selector/1
  Bus Selector/1 -> [F_Fail_Initiate]  "<F_Fail_Initiate>"
  Bus Selector/2 -> [F_Hold_Last]  "<F_Hold_Last>"
  Product14/1 -> Relational Operator1/1, Relational Operator/1, Saturation/2  "pos"
  Saturation/1 -> For Each Subsystem/2(pos_in), Sum/1  "pos_lim"
  Integrator/1 -> Sum2/2
  [F_Hold_Last] -> Product5/2
  For Each Subsystem/1(pos) -> Product16/1
  Sum1/1 -> Rate Sat/2  "Ydot"
  Product1/1 -> Sum1/1
  Bus Selector/5 -> [F_Pos_Bias]  "<F_Pos_Bias>"
  Bus Selector/10 -> [F_Rate_Scale]  "<F_Rate_Scale>"
  Bus Selector/9 -> [F_Rate_Bias]  "<F_Rate_Bias>"
  Bus Selector/13 -> Terminator2/1  "<F_Accel_Bias>"
  Bus Selector/14 -> Terminator3/1  "<F_Accel_Scale>"
  Product5/1 -> For Each Subsystem/1(Cont_Switch)
  [F_Fail_Initiate] -> Product5/1
  Bus Selector/15 -> Terminator/1  "<F_Up_Alim>"
  Bus Selector/16 -> Terminator1/1  "<F_Lwr_Alim>"
  Bus Selector/7 -> [F_Up_Plim]  "<F_Up_Plim>"
  Bus Selector/8 -> [F_Lwr_Plim]  "<F_Lwr_Plim>"
  Bus Selector/11 -> [F_Up_Rlim]  "<F_Up_Rlim>"
  Bus Selector/12 -> [F_Lwr_Rlim]  "<F_Lwr_Rlim>"
  [F_Up_Rlim] -> Rate Sat/1
  [F_Lwr_Rlim] -> Rate Sat/3
  [F_Up_Plim] -> Saturation/1
  [F_Lwr_Plim] -> Saturation/3
  Sum2/1 -> Product14/1  "pos"
  Bus Selector/6 -> [F_Pos_Scale]  "<F_Pos_Scale>"
  [F_Post_Scale] -> Product16/2
  Product16/1 -> POS/1  "pos"
  [F_Pre_Scale] -> Product18/2
  Product18/1 -> Sum/2
  Bus Selector/4 -> [F_Post_Scale]  "<F_Post_Scale>"
  Bus Selector/3 -> [F_Pre_Scale]  "<F_Pre_Scale>"
  [F_Rate_Bias] -> Sum1/2
  [F_Rate_Scale] -> Product1/1
  [F_Pos_Bias] -> Sum2/1
  [F_Pos_Scale] -> Product14/2
  [F_Up_Plim] -> Relational Operator/2
  [F_Lwr_Plim] -> Relational Operator1/2
  Relational Operator/1 -> Logical Operator5/1
  Relational Operator1/1 -> Logical Operator5/2
  Logical Operator5/1 -> Product/1
